simulink model "CAN231"  (Simulink 6.4)
settings: Solver=FixedStepDiscrete  StartTime=0.0  StopTime=inf  FixedStep=0.001  RelTol=1e-3
libraries: dsPICdrivers x11, simulink x3
settings Model: Creator=just4you  LastModifiedBy=Administrateur
settings OptimizationCC: InlineParams=on  OptimizeModelRefInitCode=on  LifeSpan=1
settings DebuggingCC: SignalResolutionControl=UseLocalSettings  StrictBusMsg=None
settings HardwareCC: ProdBitPerInt=16  ProdEndianess=LittleEndian  ProdWordSize=16  ProdHWDeviceType=16-bit Generic  TargetHWDeviceType=32-bit Generic
settings RTWCC: SystemTargetFile=dspic.tlc  TemplateMakefile=dspic_pic30_gcc.tmf  PostCodeGenCommand=dsPIC_Compile()  Description=Embedded Target for Microchip dsPIC (real-time)  GenerateReport=on  ProcessScript=dspic_make_rtw_hook  IncludeHyperlinkInReport=on  LaunchReport=on
settings CodeAppCC: IgnoreCustomStorageClasses=off
settings STFCustomTargetCC: TargetFcnLib=ansi_tfl_tmw.mat  GenFloatMathFcnCalls=ANSI_C  ModelReferenceCompliant=off  IncludeMdlTerminateFcn=off  CombineOutputUpdateFcns=on  SuppressErrorStatus=on  ERTCustomFileBanners=on  SupportContinuousTime=off  SupportNonInlinedSFcns=off  SystemTargetFile=dspic.tlc
settings ERTTargetCC: TargetFcnLib=ansi_tfl_tmw.mat  GenFloatMathFcnCalls=ANSI_C  ModelReferenceCompliant=off  ParMdlRefBuildCompliant=off  CompOptLevelCompliant=off  IncludeMdlTerminateFcn=off  SuppressErrorStatus=on  ModelStepFunctionPrototypeControlCompliant=off  InlinedParameterPlacement=NonHierarchical  ERTSrcFileBannerTemplate=dsPIC_code_template.cgt  ERTHdrFileBannerTemplate=dsPIC_code_template.cgt  ERTDataSrcFileTemplate=dsPIC_code_template.cgt  ERTDataHdrFileTemplate=dsPIC_code_template.cgt  ERTCustomFileTemplate=dsPIC_main.tlc
settings CustomProperty: DataType=string  Value=C:\PROGRA~1\MATLAB\R2009a\bin\win32\gmake

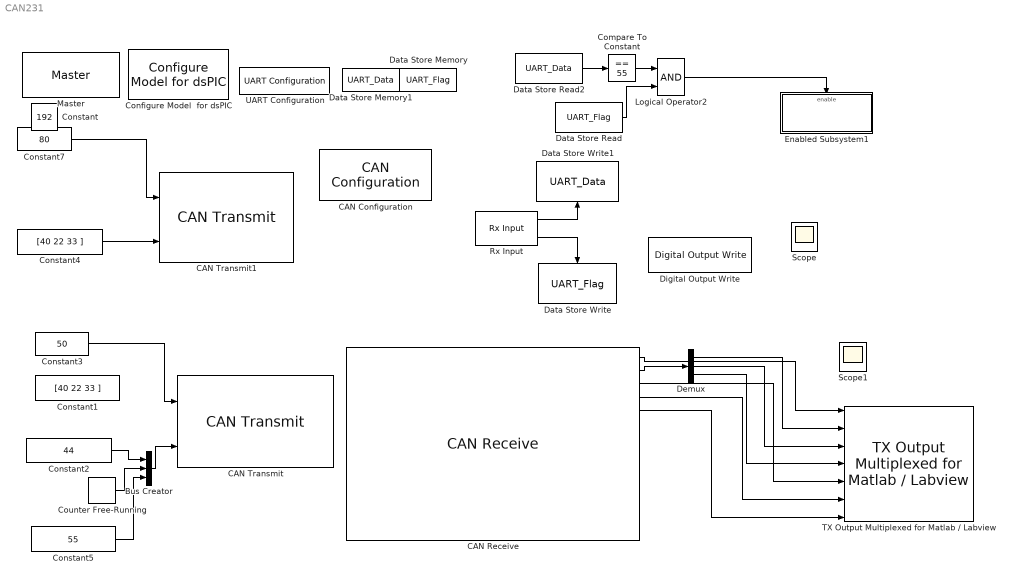
== system CAN231 ==
  Bus Creator : BusCreator  Inputs=3
  CAN Configuration : dsPICdrivers/BUS CAN/CAN Configuration  Tag=dsPIC_CAN_Config  NumCAN=1  Mode=Loop back  TcanTcy=Tcan = Tcy  BRP=34  PRSEG=1  SEG1PH=3  SAM_popup=Once at sample point  SEG2PH=3  SJW=2  SampleTime=-1  OrderingInOutPopup=None  Info="Tq = 3.5e-006s   X 9  -->  Fcan = 31.746 KHz"
  CAN Receive : dsPICdrivers/BUS CAN/CAN Receive  Tag=dsPIC_CAN_Receive  NumCAN=1  RXM0=2^29-1  DL0=3  RXF0=51  F0type=Standard or Extended  DL0received=on  FlagNewMessage0=on  OutId0=on  DataRequestSend0=on  DL1=3  RXF1=72  F1type=Standard 11 bits  DL1received=off  FlagNewMessage1=off  OutId1=off  DataRequestSend1=off  RXM1=2^11-1  DL2=4  RXF2=826  F2type=Standard or Extended  DL2received=on  FlagNewMessage2=on  OutId2=on  DataRequestSend2=on  DL3=Off  RXF3=0  F3type=Standard or Extended  DL3received=off  FlagNewMessage3=off  OutId3=off  DataRequestSend3=off  DL4=Off  RXF4=0  F4type=Standard or Extended  DL4received=off  FlagNewMessage4=off  OutId4=off  DataRequestSend4=off  DBEN=off  ErrCount=on  DataLost=on  SampleTime=-1  OrderingInOutPopup=None  Info=0
  CAN Transmit : dsPICdrivers/BUS CAN/CAN Transmit  Tag=dsPIC_CAN_Transmit  NumCAN=1  WaitPreviousTransmission=off  TxPriority=Highest  IdentifierType=Extended 29 bits  IdentifierBlockInput=on  Identifier=0  SRR=Normal Message  DLC=3  TransmitBlockInput=on  TransmitValue=0  TxFull=on  OutErrCount=on  TXBO=on  TXEP=on  TXWAR=on  SampleTime=-1  OrderingInOutPopup=Output  Info=0
  CAN Transmit1 : dsPICdrivers/BUS CAN/CAN Transmit  Tag=dsPIC_CAN_Transmit  NumCAN=1  WaitPreviousTransmission=off  TxPriority=Highest  IdentifierType=Extended 29 bits  IdentifierBlockInput=on  Identifier=0  SRR=Normal Message  DLC=3  TransmitBlockInput=on  TransmitValue=0  TxFull=on  OutErrCount=on  TXBO=on  TXEP=on  TXWAR=on  SampleTime=-1  OrderingInOutPopup=Output  Info=0
  Compare To Constant : simulink/Logic and Bit Operations/Compare To Constant  SystemSampleTime=-1  relop===  const=55  LogicOutDataTypeMode=boolean  ZeroCross=off
  Configure Model  for dsPIC : dsPICdrivers/Simulink Configuration/Configure Model  for dsPIC
  Constant1 : Constant  Value=[40 22 33 ]  OutDataTypeMode=uint8  OutDataType=sfix(16)  OutScaling=2^0  SampleTime=.01
  Constant2 : Constant  Value=44  OutDataTypeMode=uint8  OutDataType=sfix(16)  OutScaling=2^0  SampleTime=.5
  Constant3 : Constant  Value=50  OutDataType=sfix(16)  OutScaling=2^0  SampleTime=.5
  Constant4 : Constant  Value=[40 22 33 ]  OutDataTypeMode=uint8  OutDataType=sfix(16)  OutScaling=2^0  SampleTime=-1
  Constant5 : Constant  Value=55  OutDataTypeMode=uint8  OutDataType=sfix(16)  OutScaling=2^0  SampleTime=-1
  Constant7 : Constant  Value=80  OutDataType=sfix(16)  OutScaling=2^0  SampleTime=.1
  Counter Free-Running : simulink/Sources/Counter Free-Running  SystemSampleTime=-1  NumBits=8  tsamp=-1
  Data Store Memory : DataStoreMemory  DataStoreName=UART_Flag  ReadBeforeWriteMsg=warning  WriteAfterWriteMsg=warning  WriteAfterReadMsg=warning  OutDataType=sfix(16)  OutScaling=2^0
  Data Store Memory1 : DataStoreMemory  DataStoreName=UART_Data  ReadBeforeWriteMsg=warning  WriteAfterWriteMsg=warning  WriteAfterReadMsg=warning  OutDataType=sfix(16)  OutScaling=2^0
  Data Store Read : DataStoreRead  DataStoreName=UART_Flag  SampleTime=-1
  Data Store Read2 : DataStoreRead  DataStoreName=UART_Data  SampleTime=.01
  Data Store Write : DataStoreWrite  Orientation=down  DataStoreName=UART_Flag  SampleTime=-1
  Data Store Write1 : DataStoreWrite  Orientation=up  DataStoreName=UART_Data  SampleTime=-1
  Demux : Demux  Outputs=3
  Digital Output Write : dsPICdrivers/Digital I//O/Digital Output Write  Tag=dsPIC_Digital_Output  Priority=5  PORT=F  Simultaneous=off  OrderingInOutPopup=None
  Enabled Subsystem1 : Subsystem  TreatAsAtomicUnit=on
  Logical Operator2 : Logic  AllPortsSameDT=off  OutDataTypeMode=boolean
  Master : dsPICdrivers/Master  Tag=dsPIC_MASTER  Priority=1  TimeStepType=Timer1  picType=30f4012  fcy=20e6  Quartz_33f=10e6  PLLActive_33f=off  fcyDesired_33f=40e6  tmr1="[1  19999  0]"  tmr1Info="Time Step : 0.001  ;   Error : 0%  PR1=19999"  tmr2345="[0  0  0  0]"  tmr2345cfg=[-1 -1 -1 -1]  IOautoConf=on  typePort="[ 0   0   0   0   0   0   0   0   0   0   0   0   0   0   0   0   0   0   0   0   0   0   0   0   0   0   0   0   0   0   0   0   0   0   0   0   0   0   0   0   0   0   0   0   0   5   4   0   0   0   0   0   0   0   0   0   0   0   0   0   0   0   0   0   0   0   0   0   0   0   0   0   0   0   0   0   0   0   0   0   0   0   0  10   0   0   0   0   0   0   0   0   0   0   0   0   0   0   0   0   0   0   0   0   0   0   0   0   0   0   0   0 ]"  TRIS="[ 65535  65535  65535  65535  65535  65527  65535 ]"  ADPCFG=0  MasterBusyPort=None  MasterOverloadPort=None  FOSC=XT_PLL8  ClockSwitchMonitor=Both disabled  TempProtection_33f=TEMP_ON  FPBOR=PBOR_OFF  PWRT=PWRT_OFF  MCLR=MCLR_DIS  PowerSave=off  OverrideFcy=off  NewFcy=1e6  PR2345="[65535  65535  65535  65535]"
  Rx Input : dsPICdrivers/Serial PORT/Rx Input  Tag=dsPIC_RX  Priority=5  UART=1  SampleTime=.01  BlockingFctChk=off  OutputDefault=0  IsPresentFlagChk=on
  Scope : Scope
  Scope1 : Scope
  TX Output Multiplexed for Matlab / Labview : dsPICdrivers/Serial PORT/TX Output Multiplexed for Matlab // Labview  Tag=dsPIC_TX_Multiplexed  Priority=5  UART=1  CleverSpreadingChk=on  CleverSpreading=1  CHANNEL=[0 1 2 3 4 5 6 ]  CHANNELBLOCKED=[]  CHANNELBLOCKED_BITEWISE=0  Status=OK
  UART Configuration : dsPICdrivers/Serial PORT/UART Configuration  Tag=dsPIC_config_UART  Priority=2  UART=1  proposed_BAUD=115200  ALT_TX_RX=on  InterruptTxWhen=When Transmit Buffer is empty  TXInterruptPri=5  TxBufferSize=32  TXEN=on  InterruptRxWhen=When Receive Buffer is full (contain 4 characters)  RXInterruptPri=1  RxBufferSize=32  BAUD=115200  UxBRG=10  Info="UxBRG = 10   ||  Real Baud : 113636   ||  % error : -1.3573  ||  max 11.3636 Bytes / Step"  RealBaud=0
  Constant : Constant  Tag=dsPIC_CAN_Receive  IOType=siggen  Value=192  OutDataTypeMode=uint8  OutDataType=sfix(16)  OutScaling=2^0
  wires:
  Rx Input/2 -> Data Store Write/1
  Rx Input/1 -> Data Store Write1/1
  Compare To Constant/1 -> Logical Operator2/1
  Logical Operator2/1 -> Enabled Subsystem1/Enable
  Data Store Read/1 -> Logical Operator2/2
  Data Store Read2/1 -> Compare To Constant/1
  Constant3/1 -> CAN Transmit/1
  CAN Receive/1 -> TX Output Multiplexed for Matlab / Labview/1
  Constant2/1 -> Bus Creator/1
  Counter Free-Running/1 -> Bus Creator/2
  Constant5/1 -> Bus Creator/3
  Bus Creator/1 -> CAN Transmit/2
  CAN Receive/2 -> Demux/1
  Demux/1 -> TX Output Multiplexed for Matlab / Labview/2
  Demux/2 -> TX Output Multiplexed for Matlab / Labview/3
  Demux/3 -> TX Output Multiplexed for Matlab / Labview/4
  CAN Receive/3 -> TX Output Multiplexed for Matlab / Labview/5
  CAN Receive/4 -> TX Output Multiplexed for Matlab / Labview/6
  CAN Receive/5 -> TX Output Multiplexed for Matlab / Labview/7
  Constant7/1 -> CAN Transmit1/1
  Constant4/1 -> CAN Transmit1/2

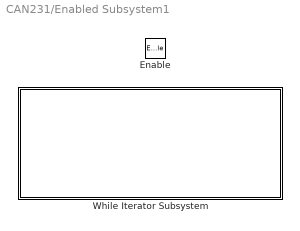
== system CAN231/Enabled Subsystem1 ==
  Enable : EnablePort
  While Iterator Subsystem : Subsystem  TreatAsAtomicUnit=on

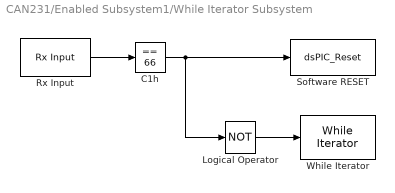
== system CAN231/Enabled Subsystem1/While Iterator Subsystem ==
  C1h : simulink/Logic and Bit Operations/Compare To Constant  SystemSampleTime=-1  relop===  const=66  LogicOutDataTypeMode=boolean  ZeroCross=off
  Logical Operator : Logic  Operator=NOT  AllPortsSameDT=off  OutDataTypeMode=boolean
  Rx Input : dsPICdrivers/Serial PORT/Rx Input  Tag=dsPIC_RX  Priority=5  UART=1  SampleTime=-1  BlockingFctChk=off  OutputDefault=0  IsPresentFlagChk=off
  Software RESET : S-Function  Tag=dsPIC_Reset  FunctionName=dsPIC_Reset  EnableBusSupport=off
      mask Description: Reset the microcontroller when input is different from 0
      mask Display:
      | fprintf('Reset');
      | port_label('input', 1 ,'~=0');
  While Iterator : WhileIterator  MaxIters=-1  WhileBlockType=do-while  ResetStates=reset
  wires:
  Logical Operator/1 -> While Iterator/1
  Rx Input/1 -> C1h/1
  C1h/1 -> Software RESET/1, Logical Operator/1
